simulink model "ModelBoostPFCController"  (R2026a)
settings: Solver=ode23t  StopTime=0.02  MaxStep=1e-5  AbsTol=1e-3
PreLoadFcn:
  | BoostPFCDefaultInputParameters;
model workspace (MAT data in the model file):
  ConverterKey = "BoostPFC"
undefined symbols (not defined in the file or in its folder): boostPFCController, boostPFCDesign, Vref
libraries: fl_lib x27, ee_lib x14, nesl_utility x14, ConverterLibrary x1
(part 1 of 2)
settings Model: SimulationMode=accelerator  Creator=vsolaise  LastModifiedBy=vsolaise
settings SimscapeCC: SimscapeNominalValues="[{\"value\":\"1\",\"unit\":\"A\"},{\"value\":\"1\",\"unit\":\"bar\"},{\"value\":\"1\",\"unit\":\"cm^2\"},{\"value\":\"1\",\"unit\":\"cm^3/s\"},{\"value\":\"1\",\"unit\":\"kJ/kg\"},{\"value\":\"1\",\"unit\":\"kW\"},{\"value\":\"1\",\"unit\":\"l\"},{\"value\":\"1\",\"unit\":\"N\"},{\"value\":\"1\",\"unit\":\"N*m\"},{\"value\":\"1\",\"unit\":\"V\"}]"  SimscapeLogDataHistory=5000.0

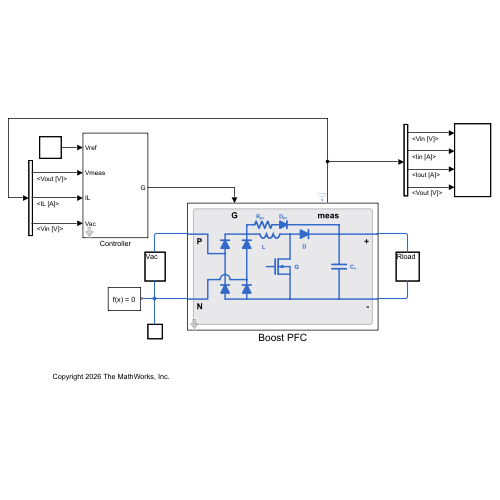
[thumbnail: Simulink's stored preview of the top-level diagram]
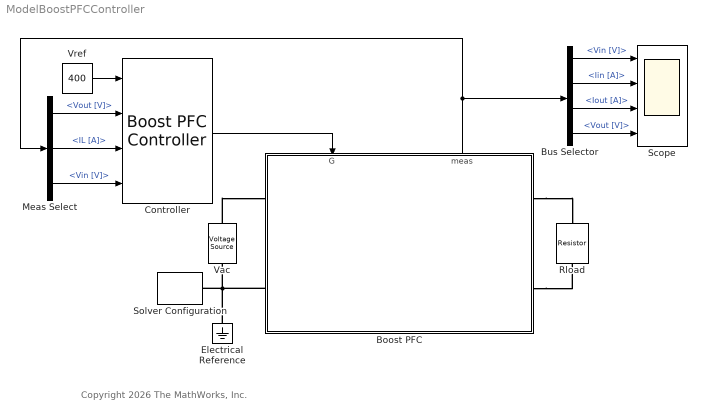
== system ModelBoostPFCController ==
  note: Copyright 2026 The MathWorks, Inc.
  Boost PFC : Subsystem  mask(Boost PFC Converter){modelOption=Simplified, ratedPower=boostPFCDesign.ratedPower.value, ratedPower_unit=W, VIn=boostPFCDesign.nomInputVoltage.value, VIn_unit=V, FRated=boostPFCDesign.lineFrequency.value, FRated_unit=Hz, VOut=boostPFCDesign.outputVoltage.value, VOut_unit=V, Fsw=boostPFCDesign.switchingFrequency.value, Fsw_unit=Hz, LBoost=boostPFCDesign.boostInductance.value, LBoost_unit=H, RLboost=boostPFCDesign.inductorResistance.value, RLboost_unit=Ohm, CBoost=2*boostPFCDesign.outputCapacitance.value, CBoost_unit=F, Rco=boostPFCDesign.capacitorResistance.value, Rco_unit=Ohm, Vco=Vref*0.95, Vco_unit=V, switchDeviceOption=MOSFET (Ideal, Switching) with Thermal, RdsOn=0.05, RdsOn_unit=Ohm, GdsOff=1e-5, GdsOff_unit=1/Ohm, Vth=3, Vth_unit=V, diodeDeviceOption=Tabulated Diode, VfDiode=0.6, VfDiode_unit=V, RdDiode=0.01, RdDiode_unit=Ohm, GdDiode=1e-5, GdDiode_unit=1/Ohm, rectDiodeDeviceOption=Tabulated Diode, VfRect=0.6, VfRect_unit=V, RdRect=0.3, RdRect_unit=Ohm, GdRect=1e-5, GdRect_unit=1/Ohm, VfPreCharge=0.6, VfPreCharge_unit=V, RdPreCharge=0.01, RdPreCharge_unit=Ohm, GdPreCharge=1e-5, GdPreCharge_unit=1/Ohm, RPreCharge=3, RPreCharge_unit=Ohm, simTemp=25, simTemp_unit=degC}
      mask prompts: modelOption "Boost PFC model option"; ratedPower "Rated power"; VIn "AC input voltage (RMS)"; FRated "Line frequency"; VOut "DC output voltage"; Fsw "Switching frequency"; LBoost "Boost inductance"; RLboost "Inductor resistance"; CBoost "Output capacitance"; Rco "Capacitor ESR"; Vco "Initial output capacitor voltage"; switchDeviceOption "Switch model"; RdsOn "On-state resistance"; GdsOff "Off-state conductance"; Vth "Threshold voltage"; diodeDeviceOption "Diode model"; VfDiode "Forward voltage"; RdDiode "On resistance"; GdDiode "Off conductance"; rectDiodeDeviceOption "Rectifier diode model"; VfRect "Forward voltage"; RdRect "On resistance"; GdRect "Off conductance"; VfPreCharge "Forward voltage"; RdPreCharge "On resistance"; GdPreCharge "Off conductance"; RPreCharge "Pre-charge resistance"; simTemp "Simulation temperature"
      mask help: Single-phase diode bridge + boost PFC power stage
      mask init:
      | %% Unit conversion: convert displayed values to base SI units
      | convMap = containers.Map( ...
      |     {'W','kW','MW','V','kV','mV','F','mF','uF','nF','pF', ...
      |      'H','mH','uH','nH','Ohm','kOhm','mOhm','S','mS','1/Ohm', ...
      |      'Hz','kHz','MHz'}, ...
      |     {1, 1e3, 1e6, 1, 1e3, 1e-3, 1, 1e-3, 1e-6, 1e-9, 1e-12, ...
      |      1, 1e-3, 1e-6, 1e-9, 1, 1e3, 1e-3, 1, 1e-3, 1, ...
      |      1, 1e3, 1e6});
      | 
      | ratedPower_SI = ratedPower * convMap(ratedPower_unit);
      | VIn_SI = VIn * convMap(VIn_unit);
      | FRated_SI = FRated * convMap(FRated_unit);
      | VOut_SI = VOut * convMap(VOut_unit);
      | Fsw_SI = Fsw * convMap(Fsw_unit);
      | LBoost_SI = LBoost * convMap(LBoost_unit);
      | RLboost_SI = RLboost * convMap(RLboost_unit);
      | CBoost_SI = CBoost * convMap(CBoost_unit);
      | Rco_SI = Rco * convMap(Rco_unit);
      | Vco_SI = Vco * convMap(Vco_unit);
      | RdsOn_SI = RdsOn * convMap(RdsOn_unit);
      | GdsOff_SI = GdsOff * convMap(GdsOff_unit);
      | Vth_SI = Vth * convMap(Vth_unit);
      | VfDiode_SI = VfDiode * convMap(VfDiode_unit);
      | RdDiode_SI = RdDiode * convMap(RdDiode_unit);
      | GdDiode_SI = GdDiode * convMap(GdDiode_unit);
      | 
      | 
      | VfRect_SI = VfRect * convMap(VfRect_unit);
      | RdRect_SI = RdRect * convMap(RdRect_unit);
      | GdRect_SI = GdRect * convMap(GdRect_unit);
      | % Pre-charge circuit parameters
      | VfPreCharge_SI = VfPreCharge * convMap(VfPreCharge_unit);
      | RdPreCharge_SI = RdPreCharge * convMap(RdPreCharge_unit);
      | GdPreCharge_SI = GdPreCharge * convMap(GdPreCharge_unit);
      | RPreCharge_SI = RPreCharge * convMap(RPreCharge_unit);
      | 
      | 
      | %% Simulation temperature (thermal MOSFET and tabulated diodes)
      | % Temperature is an OFFSET unit (K = degC + 273.15), so it cannot use the
      | % multiplicative convMap above; convert it explicitly. simTemp_K is read directly by
      | % the thermal MOSFET junction-temperature target, by the boost switch's Temperature Source, and by
      | % every tabulated diode's device simulation temperature.
      | if strcmp(simTemp_unit, 'degC')
      |     simTemp_K = simTemp + 273.15;
      | else
      |     simTemp_K = simTemp;
      | end
      | 
      | %% Apply variant selection
      | selectBoostPFCModelOption(gcb);
      settings: CopyFcn="set_param(gcbh,\"LinkStatus\",\"none\");"  PortSchema="{\"entries\":[{\"content\":{\"sides\":[{\"content\":{\"connectorIds\":[\"LConn1\",\"LConn2\"]},\"type\":\"ConnectorPlacement.EquallySpacedRectSide\",\"uuid\":\"1dbc8d27-ad96-467a-a357-3fb6b54f5038\"},{\"content\":{\"connectorIds\":[\"RConn1\",\"RConn2\"],\"side\":\"RIGHT\"},\"type\":\"ConnectorPlacement.EquallySpacedRectSide\",\"uuid\":\"a7801564-f46e-4876-bbd0-388b36974b7d\"},{\"content\":{\"connectorIds\":[\"In1\",\"Out1\"],\"side\":\"TOP\"},\"type\":\"ConnectorPlacement.EquallySpacedRectSide\",\"uuid\":\"b9e6132f-a5e8-4db3-b298-fdce73dc02b1\"}]},\"type\":\"ConnectorPlacement.EquallySpacedConnector\",\"uuid\":\"f45ea93c-581d-4ac6-a344-7b31d290ff6c\"}],\"packageUris\":[\"http://schema.mathworks.com/mf0/Connector/R2020b\"],\"version\":\"1.0\"}"
      mask Help: web('BoostPFC.html')
      mask TypeOptions modelOption: Simplified | Detailed
      mask Callback modelOption: selectBoostPFCModelOption(gcb);
      mask TypeOptions ratedPower_unit: W | kW | MW
      mask TypeOptions VIn_unit: V | kV | mV
      mask TypeOptions FRated_unit: Hz | kHz
      mask TypeOptions VOut_unit: V | kV | mV
      mask TypeOptions Fsw_unit: Hz | kHz | MHz
      mask TypeOptions LBoost_unit: H | mH | uH
      mask TypeOptions RLboost_unit: Ohm | kOhm | mOhm
      mask TypeOptions CBoost_unit: F | mF | uF | nF
      mask TypeOptions Rco_unit: Ohm | kOhm | mOhm
      mask TypeOptions Vco_unit: V | kV | mV
      mask TypeOptions switchDeviceOption: Ideal Switch | MOSFET (Ideal, Switching) with Thermal
      mask Callback switchDeviceOption: selectBoostPFCSwitchDevice(gcb);
      mask TypeOptions RdsOn_unit: Ohm | kOhm | mOhm
      mask TypeOptions GdsOff_unit: 1/Ohm | S | mS
      mask TypeOptions Vth_unit: V | kV | mV
      mask TypeOptions diodeDeviceOption: Ideal Diode | Tabulated Diode
      mask Callback diodeDeviceOption: selectBoostPFCDiodeDevice(gcb);
      mask TypeOptions VfDiode_unit: V | kV | mV
      mask TypeOptions RdDiode_unit: Ohm | kOhm | mOhm
      mask TypeOptions GdDiode_unit: 1/Ohm | S | mS
      mask TypeOptions rectDiodeDeviceOption: Ideal Diode | Tabulated Diode
      mask Callback rectDiodeDeviceOption: selectBoostPFCRectifierDiodeDevice(gcb);
      mask TypeOptions VfRect_unit: V | mV | kV
      mask TypeOptions RdRect_unit: Ohm | mOhm | kOhm
      mask TypeOptions GdRect_unit: 1/Ohm
      mask TypeOptions VfPreCharge_unit: V | kV | mV
      mask TypeOptions RdPreCharge_unit: Ohm | kOhm | mOhm
      mask TypeOptions GdPreCharge_unit: 1/Ohm | S | mS
      mask TypeOptions RPreCharge_unit: Ohm | kOhm | mOhm
      mask TypeOptions simTemp_unit: degC | K
      mask DialogControl BoostPFCConverterParameters Prompt: Boost PFC Converter Parameters
      mask DialogControl SwitchDevice Prompt: Boost Stage Devices
      mask DialogControl openMOSFETMask Prompt: Open MOSFET block mask
      mask DialogControl openMOSFETMask Callback: open_system([gcb '/BoostPFCVariant/DetailedModel/BoostSwitch/SwitchingMOSFETwithThermal/MOSFET'], 'mask');
      mask DialogControl DiodeDevice Prompt: Boost Diode Device
      mask DialogControl openDiodeMask Prompt: Open Diode block mask
      mask DialogControl openDiodeMask Callback: open_system([gcb '/BoostPFCVariant/DetailedModel/BoostDiode/TabulatedDiode/Diode1'], 'mask');
      mask DialogControl RectifierDevices Prompt: Rectifier Devices
      mask DialogControl openRectDiodeMask Prompt: Open Rectifier Diode Mask
      mask DialogControl openRectDiodeMask Callback: open_system([gcb '/BoostPFCVariant/DetailedModel/RectifierBridge/TabulatedDiode/Diode1'], 'mask');
      mask DialogControl applyRectDiodeParam Prompt: Apply to All Rectifier Diodes
      mask DialogControl applyRectDiodeParam Callback: applyBoostPFCRectifierDiodeParameters(gcb);
      mask DialogControl PreChargeCircuit Prompt: Pre-Charge Circuit Parameters
      mask DialogControl ExportPanel Prompt: Export to Unmasked Subsystem
      mask DialogControl ExportInfo Prompt: To customize the converter, export it as an unmasked subsystem with the active variant flattened - a standalone, fully-editable circuit plus a parameter file. Requires the "Variant Manager for Simulink" add-on.
      mask DialogControl exportToModel Prompt: Export
      mask DialogControl exportToModel Callback: exportConverterModelFromMask(gcb);
      mask Display: image('BoostPFCDiodeIcon.svg');
  Bus Selector : BusSelector  OutputSignals=Vin [V],Iin [A],Iout [A],Vout [V]
  Controller : ConverterLibrary/Controller/Power Factor Correction Converters/Boost PFC Controller  outputSelect=PWM Signal  cntrlSelect=PI controller (Continuous)  VacRMS=boostPFCDesign.nomInputVoltage.value  VbaseDC=boostPFCDesign.outputVoltage.value  Pbase=boostPFCDesign.ratedPower.value  PrefPu=boostPFCController.PrefPu  iRefPeakMaxPu=boostPFCController.iRefPeakMaxPu  Fsw=boostPFCDesign.switchingFrequency.value  Ts=boostPFCController.TsPwm  gateVoltageOn=boostPFCController.gateVoltageOn  gateVoltageOff=boostPFCController.gateVoltageOff  KpVoltage=boostPFCController.KpVoltage  KiVoltage=boostPFCController.KiVoltage  TsVoltage=boostPFCController.TsVoltage  KpCurrent=boostPFCController.KpCurrent  KiCurrent=boostPFCController.KiCurrent  dutyMax=boostPFCController.dutyMax  dutyMin=boostPFCController.dutyMin  TsCurrent=boostPFCController.TsCurrent
      link override Current Controller: LabelModeActiveChoice=PIContinuous
      link override Output Mode: LabelModeActiveChoice=PWMSignal
      link override Output Mode/PWMSignal/Ramp Mode: LabelModeActiveChoice=VariableStep
      link override Voltage Controller: LabelModeActiveChoice=PIContinuous
      settings: SourceProductName=Simscape Power Converter Components
  Electrical Reference : fl_lib/Electrical/Electrical Elements/Electrical Reference
  Meas Select : BusSelector  OutputSignals=Vout [V],IL [A],Vin [V]
  Rload : fl_lib/Electrical/Electrical Elements/Resistor  R=160 Ohm  i_specify=off  i_priority=None  i=0 A  i_nominal_specify=off  i_nominal_value=1  i_nominal_unit=A  v_specify=off  v_priority=None  v=0 V  v_nominal_specify=off  v_nominal_value=1  v_nominal_unit=V
  Scope : Scope  NumInputPorts=4
      settings: ActiveDisplayString=4  Title=Output Voltage (V)  ActiveDisplayYMinimum=303.40542444423374  ActiveDisplayYMaximum=409.6389638703705
  Solver Configuration : nesl_utility/Solver Configuration  PhysicalDomain=network_engine_domain  SubClassName=solver  LeftPortType=input  RightPortType=generic  Tones=[]  Harmonics=[]  SimulateNoise=off  Profile=off  UseLocalSampling=off  EnableSwitchedLinearOptims=on  FrequencyDomain=off  UseCCode=off  RelTol=0.001  AbsTol=0.001  MinStep=1e-09  ToWorkspace=off  RevertToSquareIcSolve=off  NumHomotopyIterations=100  PhasorMode=off  PhasorModeNumHarmonics=1  ConsistencySolver=NEWTON_XTOL_AFTER_FTOL  CanonicalOrdering=UNORDERED  OptimizeIntermediates=UNOPTIMIZED  IndexReductionMethod=DerivativeReplacement  DoDC=off  ResidualTolerance=1e-09  ConsistencyTolSource=GLOBAL  ConsistencyAbsTol=0.001  ConsistencyRelTol=0.001  ConsistencyTolFactor=0.001  UseLocalSolver=on  LocalSolverChoice=NE_BACKWARD_EULER_ADVANCER  ResolveIndetEquations=on  FunctionEvalNumThread=1  LocalSolverSampleTime=1/(25*boostPFCDesign.switchingFrequency.value)  DoFixedCost=off  MaxNonlinIter=3  MaxModeIter=2  ComputeImpulses=off  ImpulseIterations=2  LinearAlgebra=auto  LinearAlgebraNumThread=0  EquationFormulation=NE_TIME_EF  DelaysMemoryBudget=1024  AutomaticFiltering=on  FilteringTimeConstant=0.001  PartitionStorageMethod=AS_NEEDED  PartitionMemoryBudget=1024  PartitionMethod=ROBUST  MultibodyUseLocalSolver=off  MultibodyLocalSolverChoice=ODE1  MultibodyLocalSolverSampleTime=0.001
  Vac : ee_lib/Sources/Voltage Source  dc_voltage=0 V  ac_voltage=230*sqrt(2) V  ac_shift=0 rad  ac_frequency=50 Hz  noise_mode=ee.enum.sources.noise.Disabled  PSD=0 V^2/Hz  sample_time=1e-3 s  repeatability=ee.enum.sources.repeatability.NotRepeatable  user_seed=0  auto_seed=436666721  i_specify=off  i_priority=None  i=0 A  i_nominal_specify=off  i_nominal_value=1  i_nominal_unit=A  v_specify=off  v_priority=None  v=0 V  v_nominal_specify=off  v_nominal_value=1  v_nominal_unit=V
  Vref : Constant  Value=400
  wires:
  Boost PFC/1(meas) -> Meas Select/1, Bus Selector/1
  Vref/1 -> Controller/1
  Meas Select/1 -> Controller/2  "<Vout [V]>"
  Meas Select/2 -> Controller/3  "<IL [A]>"
  Meas Select/3 -> Controller/4  "<Vin [V]>"
  Controller/1 -> Boost PFC/1(G)
  Bus Selector/1 -> Scope/1  "<Vin [V]>"
  Bus Selector/2 -> Scope/2  "<Iin [A]>"
  Bus Selector/3 -> Scope/3  "<Iout [A]>"
  Bus Selector/4 -> Scope/4  "<Vout [V]>"
  connections:
  Vac/LConn1 -- Boost PFC/LConn1
  Boost PFC/RConn1 -- Rload/LConn1
  Boost PFC/RConn2 -- Rload/RConn1
  Electrical Reference/LConn1 -- Boost PFC/LConn2 -- Solver Configuration/RConn1 -- Vac/RConn1

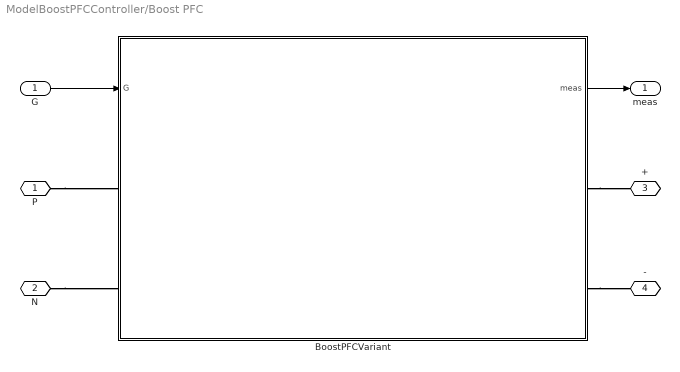
== system ModelBoostPFCController/Boost PFC ==
  G : Inport
  BoostPFCVariant : Subsystem  Variant=on  VariantControlMode=label  LabelModeActiveChoice=SimplifiedModel
  P : PMIOPort  Side=Left
  N : PMIOPort  Port=2  Side=Left
  + : PMIOPort  Port=3  Side=Right
  - : PMIOPort  Port=4  Side=Right
  meas : Outport
  wires:
  BoostPFCVariant/1(meas) -> meas/1
  G/1 -> BoostPFCVariant/1(G)
  connections:
  BoostPFCVariant/RConn2 -- -/RConn1
  BoostPFCVariant/RConn1 -- +/RConn1
  N/RConn1 -- BoostPFCVariant/LConn2
  P/RConn1 -- BoostPFCVariant/LConn1

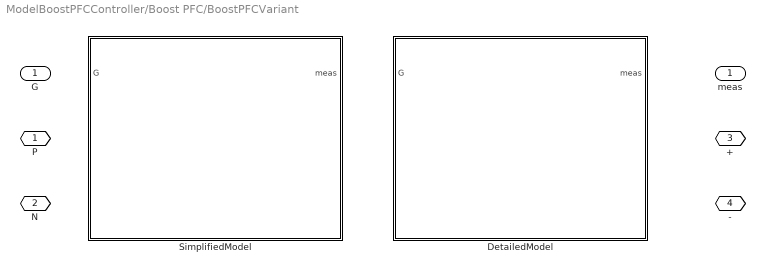
== system ModelBoostPFCController/Boost PFC/BoostPFCVariant ==
  G : Inport
  DetailedModel : Subsystem  VariantControl=DetailedModel
  SimplifiedModel : Subsystem  VariantControl=SimplifiedModel
  P : PMIOPort  Side=Left
  N : PMIOPort  Port=2  Side=Left
  + : PMIOPort  Port=3  Side=Right
  - : PMIOPort  Port=4  Side=Right
  meas : Outport

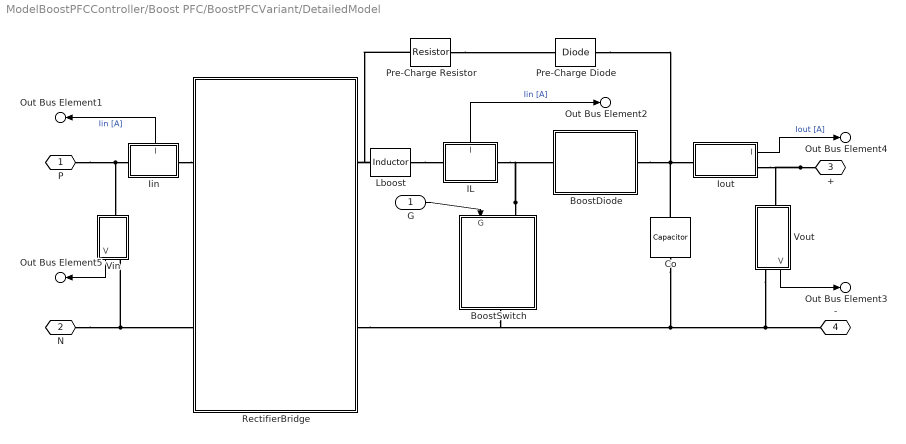
== system ModelBoostPFCController/Boost PFC/BoostPFCVariant/DetailedModel ==
  G : Inport
  BoostDiode : Subsystem  Variant=on  VariantControlMode=label  LabelModeActiveChoice=TabulatedDiode
  BoostSwitch : Subsystem  Variant=on  VariantControlMode=label  LabelModeActiveChoice=SwitchingMOSFETwithThermal
  Co : ee_lib/Passive/Capacitor  cap_option=ee.enum.passive.capacitor.capOption.const  c=CBoost_SI F  Cvec=[1e-05, 1e-06] F  Vvec=[0, 10] V  CV_table_symmetry=ee.enum.passive.capacitor.tableSymmetry.yes  f_vec=[1, 10] kHz  DFext_vec=[.8, 1.2]  enable_C_tol=ee.enum.toleranceApplication.none  averaging_period=0 s  C_tol=5  tol_distribution=ee.enum.toleranceDistribution.uniform  nSigma=4  r=Rco_SI Ohm  g=0 1/Ohm  enable_operating_limits=ee.enum.enable.no  operating_limit_action=ee.enum.passive.reportOpLim.warn  max_working_voltage_range=[-25, 25] V  power_rating=1 W  maxTemperature=85 degC  thermalEnable=false  thermalMass=1 J/K  i_specify=off  i_priority=None  i=0 A  i_nominal_specify=off  i_nominal_value=1  i_nominal_unit=A  v_specify=off  v_priority=None  v=0 V  v_nominal_specify=off  v_nominal_value=1  v_nominal_unit=V  vc_specify=on  vc_priority=High  vc=Vco_SI V  vc_nominal_specify=off  vc_nominal_value=1  vc_nominal_unit=V  T_specify=off  T_priority=None  T=298.15 K  T_nominal_specify=off  T_nominal_value=1  T_nominal_unit=K
  IL : Subsystem
      settings: PortSchema="{\"entries\":[{\"content\":{\"sides\":[{\"content\":{\"connectorIds\":[\"LConn1\"]},\"type\":\"ConnectorPlacement.EquallySpacedRectSide\",\"uuid\":\"80632e7e-66fe-49c8-894c-61cf7358e53a\"},{\"content\":{\"connectorIds\":[\"RConn1\"],\"side\":\"RIGHT\"},\"type\":\"ConnectorPlacement.EquallySpacedRectSide\",\"uuid\":\"7fb991d4-0257-47fa-8c16-238ff3f2e60c\"},{\"content\":{\"connectorIds\":[\"Out1\"],\"side\":\"TOP\"},\"type\":\"ConnectorPlacement.EquallySpacedRectSide\",\"uuid\":\"a2cf4f5e-7cb3-4577-a513-817a4fd9f07d\"}]},\"type\":\"ConnectorPlacement.EquallySpacedConnector\",\"uuid\":\"e3fac4ca-b917-4eeb-beb4-75837a4782c1\"}],\"packageUris\":[\"http://schema.mathworks.com/mf0/Connector/R2020b\"],\"version\":\"1.0\"}"
      mask Display: disp('I')
  Iin : Subsystem
      settings: PortSchema="{\"entries\":[{\"content\":{\"sides\":[{\"content\":{\"connectorIds\":[\"LConn1\"]},\"type\":\"ConnectorPlacement.EquallySpacedRectSide\",\"uuid\":\"80632e7e-66fe-49c8-894c-61cf7358e53a\"},{\"content\":{\"connectorIds\":[\"RConn1\"],\"side\":\"RIGHT\"},\"type\":\"ConnectorPlacement.EquallySpacedRectSide\",\"uuid\":\"7fb991d4-0257-47fa-8c16-238ff3f2e60c\"},{\"content\":{\"connectorIds\":[\"Out1\"],\"side\":\"TOP\"},\"type\":\"ConnectorPlacement.EquallySpacedRectSide\",\"uuid\":\"a2cf4f5e-7cb3-4577-a513-817a4fd9f07d\"}]},\"type\":\"ConnectorPlacement.EquallySpacedConnector\",\"uuid\":\"e3fac4ca-b917-4eeb-beb4-75837a4782c1\"}],\"packageUris\":[\"http://schema.mathworks.com/mf0/Connector/R2020b\"],\"version\":\"1.0\"}"
      mask Display: disp('I')
  Iout : Subsystem
      mask Display: disp('I')
  Lboost : ee_lib/Passive/Inductor  l=LBoost_SI H  enable_L_tol=ee.enum.toleranceApplication.none  L_tol=20  tol_distribution=ee.enum.toleranceDistribution.uniform  nSigma=4  r=RLboost_SI Ohm  g=1e-9 1/Ohm  enable_operating_limits=ee.enum.enable.no  operating_limit_action=ee.enum.passive.reportOpLim.warn  max_working_current=1 A  power_rating=1 W  i_L_specify=off  i_L_priority=High  i_L=0 A  i_L_nominal_specify=off  i_L_nominal_value=1  i_L_nominal_unit=A
  Pre-Charge Diode : fl_lib/Electrical/Electrical Elements/Diode  Vf=VfPreCharge_SI V  Ron=RdPreCharge_SI Ohm  Goff=GdPreCharge_SI 1/Ohm  i_specify=off  i_priority=None  i=0 A  i_nominal_specify=off  i_nominal_value=1  i_nominal_unit=A  v_specify=off  v_priority=None  v=0 V  v_nominal_specify=off  v_nominal_value=1  v_nominal_unit=V
  Pre-Charge Resistor : fl_lib/Electrical/Electrical Elements/Resistor  R=RPreCharge_SI Ohm  i_specify=off  i_priority=None  i=0 A  i_nominal_specify=off  i_nominal_value=1  i_nominal_unit=A  v_specify=off  v_priority=None  v=0 V  v_nominal_specify=off  v_nominal_value=1  v_nominal_unit=V
  RectifierBridge : Subsystem  Variant=on  VariantControlMode=label  LabelModeActiveChoice=TabulatedDiode
  Vin : Subsystem
      mask Display: disp('V')
  Vout : Subsystem
      settings: PortSchema="{\"entries\":[{\"content\":{\"sides\":[{\"content\":{\"connectorIds\":[\"LConn1\"]},\"type\":\"ConnectorPlacement.EquallySpacedRectSide\",\"uuid\":\"80632e7e-66fe-49c8-894c-61cf7358e53a\"},{\"content\":{\"connectorIds\":[\"RConn1\",\"Out1\"],\"side\":\"RIGHT\"},\"type\":\"ConnectorPlacement.EquallySpacedRectSide\",\"uuid\":\"7fb991d4-0257-47fa-8c16-238ff3f2e60c\"},{\"content\":{\"side\":\"TOP\"},\"type\":\"ConnectorPlacement.EquallySpacedRectSide\",\"uuid\":\"a2cf4f5e-7cb3-4577-a513-817a4fd9f07d\"}]},\"type\":\"ConnectorPlacement.EquallySpacedConnector\",\"uuid\":\"e3fac4ca-b917-4eeb-beb4-75837a4782c1\"}],\"packageUris\":[\"http://schema.mathworks.com/mf0/Connector/R2020b\"],\"version\":\"1.0\"}"
      mask Display: disp('V')
  P : PMIOPort  Side=Left
  N : PMIOPort  Port=2  Side=Left
  + : PMIOPort  Port=3  Side=Right
  - : PMIOPort  Port=4  Side=Right
  Out Bus Element1 : Outport  PortName=meas  Element=Iin [A]
  Out Bus Element2 : Outport  PortName=meas  Element=IL [A]
  Out Bus Element3 : Outport  PortName=meas  Element=Vout [V]
  Out Bus Element4 : Outport  PortName=meas  Element=Iout [A]
  Out Bus Element5 : Outport  PortName=meas  Element=Vin [V]
  wires:
  G/1 -> BoostSwitch/1(G)
  Iin/1(I) -> Out Bus Element1/1  "Iin [A]"
  IL/1(I) -> Out Bus Element2/1  "Iin [A]"
  Vout/1(V) -> Out Bus Element3/1
  Iout/1(I) -> Out Bus Element4/1  "Iout [A]"
  Vin/1(V) -> Out Bus Element5/1
  connections:
  Pre-Charge Resistor/RConn1 -- Pre-Charge Diode/LConn1
  P/RConn1 -- Iin/LConn1 -- Vin/LConn1
  N/RConn1 -- Vin/RConn1 -- RectifierBridge/LConn2
  Lboost/LConn1 -- Pre-Charge Resistor/LConn1 -- RectifierBridge/RConn1
  Lboost/RConn1 -- IL/LConn1
  BoostSwitch/LConn1 -- IL/RConn1 -- BoostDiode/LConn1
  BoostDiode/RConn1 -- Co/LConn1 -- Pre-Charge Diode/RConn1 -- Iout/LConn1
  +/RConn1 -- Vout/LConn1 -- Iout/RConn1
  Co/RConn1 -- -/RConn1 -- Vout/RConn1 -- RectifierBridge/RConn2 -- BoostSwitch/RConn1
  Iin/RConn1 -- RectifierBridge/LConn1

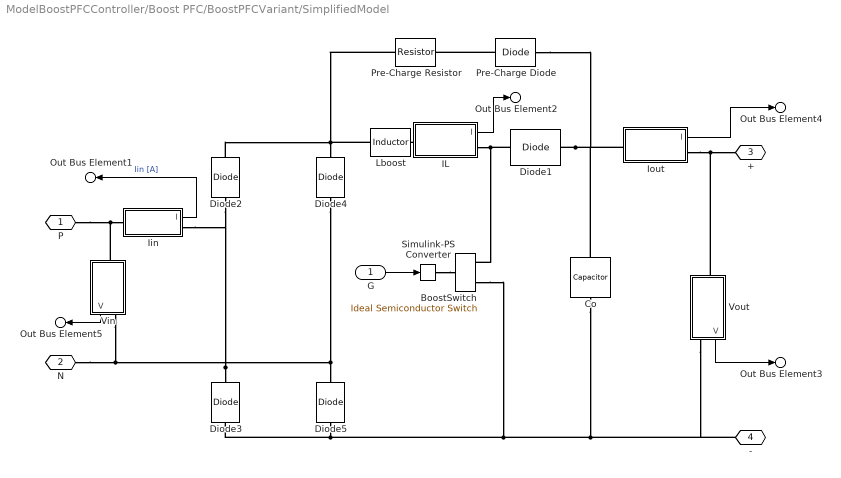
== system ModelBoostPFCController/Boost PFC/BoostPFCVariant/SimplifiedModel ==
  G : Inport
  BoostSwitch : ee_lib/Semiconductors & Converters/Ideal Semiconductor Switch  port_option=ee.enum.controlport.ps  Ron=RdsOn_SI Ohm  Goff=GdsOff_SI 1/Ohm  Vth=Vth_SI V  diode_param=ee.enum.semiconductors.protectionDiode.external  diode_Vf=0.8 V  diode_Ron=0.001 Ohm  diode_Goff=1e-5 1/Ohm  diode_C=50e-9 F  diode_iRM=-235 A  diode_iF=300 A  diode_idot=-50 A/us  diode_trr_param=ee.enum.converters.diodetrr.trr_factor  diode_trr_factor=3  diode_trr=15 us  diode_Qrr=1500 s*uA
  Co : ee_lib/Passive/Capacitor  cap_option=ee.enum.passive.capacitor.capOption.const  c=CBoost_SI F  Cvec=[1e-05, 1e-06] F  Vvec=[0, 10] V  CV_table_symmetry=ee.enum.passive.capacitor.tableSymmetry.yes  f_vec=[1, 10] kHz  DFext_vec=[.8, 1.2]  enable_C_tol=ee.enum.toleranceApplication.none  averaging_period=0 s  C_tol=5  tol_distribution=ee.enum.toleranceDistribution.uniform  nSigma=4  r=Rco_SI Ohm  g=0 1/Ohm  enable_operating_limits=ee.enum.enable.no  operating_limit_action=ee.enum.passive.reportOpLim.warn  max_working_voltage_range=[-25, 25] V  power_rating=1 W  maxTemperature=85 degC  thermalEnable=false  thermalMass=1 J/K  i_specify=off  i_priority=None  i=0 A  i_nominal_specify=off  i_nominal_value=1  i_nominal_unit=A  v_specify=off  v_priority=None  v=0 V  v_nominal_specify=off  v_nominal_value=1  v_nominal_unit=V  vc_specify=on  vc_priority=High  vc=Vco_SI V  vc_nominal_specify=off  vc_nominal_value=1  vc_nominal_unit=V  T_specify=off  T_priority=None  T=298.15 K  T_nominal_specify=off  T_nominal_value=1  T_nominal_unit=K
  Diode1 : fl_lib/Electrical/Electrical Elements/Diode  Vf=VfDiode_SI V  Ron=RdDiode_SI Ohm  Goff=GdDiode_SI 1/Ohm  i_specify=off  i_priority=None  i=0 A  i_nominal_specify=off  i_nominal_value=1  i_nominal_unit=A  v_specify=off  v_priority=None  v=0 V  v_nominal_specify=off  v_nominal_value=1  v_nominal_unit=V
  Diode{2..5} (4 alike) : fl_lib/Electrical/Electrical Elements/Diode  Vf=VfRect_SI V  Ron=RdRect_SI Ohm  Goff=GdRect_SI 1/Ohm  i_specify=off  i_priority=None  i=0 A  i_nominal_specify=off  i_nominal_value=1  i_nominal_unit=A  v_specify=off  v_priority=None  v=0 V  v_nominal_specify=off  v_nominal_value=1  v_nominal_unit=V
  IL : Subsystem
      mask Display: disp('I')
  Iin : Subsystem
      mask Display: disp('I')
  Iout : Subsystem
      mask Display: disp('I')
  Lboost : ee_lib/Passive/Inductor  l=LBoost_SI H  enable_L_tol=ee.enum.toleranceApplication.none  L_tol=20  tol_distribution=ee.enum.toleranceDistribution.uniform  nSigma=4  r=RLboost_SI Ohm  g=1e-9 1/Ohm  enable_operating_limits=ee.enum.enable.no  operating_limit_action=ee.enum.passive.reportOpLim.warn  max_working_current=1 A  power_rating=1 W  i_L_specify=off  i_L_priority=High  i_L=0 A  i_L_nominal_specify=off  i_L_nominal_value=1  i_L_nominal_unit=A
  Pre-Charge Diode : fl_lib/Electrical/Electrical Elements/Diode  Vf=VfPreCharge_SI V  Ron=RdPreCharge_SI Ohm  Goff=GdPreCharge_SI 1/Ohm  i_specify=off  i_priority=None  i=0 A  i_nominal_specify=off  i_nominal_value=1  i_nominal_unit=A  v_specify=off  v_priority=None  v=0 V  v_nominal_specify=off  v_nominal_value=1  v_nominal_unit=V
  Pre-Charge Resistor : fl_lib/Electrical/Electrical Elements/Resistor  R=RPreCharge_SI Ohm  i_specify=off  i_priority=None  i=0 A  i_nominal_specify=off  i_nominal_value=1  i_nominal_unit=A  v_specify=off  v_priority=None  v=0 V  v_nominal_specify=off  v_nominal_value=1  v_nominal_unit=V
  Simulink-PS Converter : nesl_utility/Simulink-PS Converter  PhysicalDomain=network_engine_domain  SubClassName=ps_input  LeftPortType=input  RightPortType=output  PseudoPeriodic=off  Frequencies=[]  NoiseDistribution=none  NoiseParameters=[]  Unit=1  AffineConversion=off  FilteringAndDerivatives=provide  SimscapeFilterOrder=1  InputFilterTimeConstant=0.001  UdotUserProvided=0
  Vin : Subsystem
      settings: PortSchema="{\"entries\":[{\"content\":{\"sides\":[{\"content\":{\"connectorIds\":[\"LConn1\"]},\"type\":\"ConnectorPlacement.EquallySpacedRectSide\",\"uuid\":\"5f92137b-4b58-46b8-a68f-d3527484291c\"},{\"content\":{\"connectorIds\":[\"RConn1\",\"Out1\"],\"side\":\"RIGHT\"},\"type\":\"ConnectorPlacement.EquallySpacedRectSide\",\"uuid\":\"154b36f0-aa4a-4375-80c2-9c55af429c32\"},{\"content\":{\"side\":\"TOP\"},\"type\":\"ConnectorPlacement.EquallySpacedRectSide\",\"uuid\":\"6e01dd2b-817e-4c7e-a9bf-e017a248a3a8\"}]},\"type\":\"ConnectorPlacement.EquallySpacedConnector\",\"uuid\":\"a9d15cc4-68aa-466b-9599-7a273210f999\"}],\"packageUris\":[\"http://schema.mathworks.com/mf0/Connector/R2020b\"],\"version\":\"1.0\"}"
      mask Display: disp('V')
  Vout : Subsystem
      settings: PortSchema="{\"entries\":[{\"content\":{\"sides\":[{\"content\":{\"connectorIds\":[\"LConn1\"]},\"type\":\"ConnectorPlacement.EquallySpacedRectSide\",\"uuid\":\"5f92137b-4b58-46b8-a68f-d3527484291c\"},{\"content\":{\"connectorIds\":[\"RConn1\",\"Out1\"],\"side\":\"RIGHT\"},\"type\":\"ConnectorPlacement.EquallySpacedRectSide\",\"uuid\":\"154b36f0-aa4a-4375-80c2-9c55af429c32\"},{\"content\":{\"side\":\"TOP\"},\"type\":\"ConnectorPlacement.EquallySpacedRectSide\",\"uuid\":\"6e01dd2b-817e-4c7e-a9bf-e017a248a3a8\"}]},\"type\":\"ConnectorPlacement.EquallySpacedConnector\",\"uuid\":\"a9d15cc4-68aa-466b-9599-7a273210f999\"}],\"packageUris\":[\"http://schema.mathworks.com/mf0/Connector/R2020b\"],\"version\":\"1.0\"}"
      mask Display: disp('V')
  P : PMIOPort  Side=Left
  N : PMIOPort  Port=2  Side=Left
  + : PMIOPort  Port=3  Side=Right
  - : PMIOPort  Port=4  Side=Right
  Out Bus Element1 : Outport  PortName=meas  Element=Iin [A]
  Out Bus Element2 : Outport  PortName=meas  Element=IL [A]
  Out Bus Element3 : Outport  PortName=meas  Element=Vout [V]
  Out Bus Element4 : Outport  PortName=meas  Element=Iout [A]
  Out Bus Element5 : Outport  PortName=meas  Element=Vin [V]
  wires:
  Vin/1(V) -> Out Bus Element5/1
  IL/1(I) -> Out Bus Element2/1
  Vout/1(V) -> Out Bus Element3/1
  Iout/1(I) -> Out Bus Element4/1
  Iin/1(I) -> Out Bus Element1/1  "Iin [A]"
  G/1 -> Simulink-PS Converter/1
  connections:
  Pre-Charge Diode/LConn1 -- Pre-Charge Resistor/RConn1
  Iin/LConn1 -- Vin/LConn1 -- P/RConn1
  Diode2/RConn1 -- Lboost/LConn1 -- Pre-Charge Resistor/LConn1 -- Diode4/RConn1
  Diode3/RConn1 -- Iin/RConn1 -- Diode2/LConn1
  Vin/RConn1 -- Diode4/LConn1 -- Diode5/RConn1 -- N/RConn1
  Diode5/LConn1 -- Vout/RConn1 -- -/RConn1 -- Co/RConn1 -- BoostSwitch/RConn2 -- Diode3/LConn1
  Diode1/LConn1 -- IL/RConn1 -- BoostSwitch/RConn1
  Simulink-PS Converter/RConn1 -- BoostSwitch/LConn1
  Diode1/RConn1 -- Co/LConn1 -- Pre-Charge Diode/RConn1 -- Iout/LConn1
  IL/LConn1 -- Lboost/RConn1
  Iout/RConn1 -- Vout/LConn1 -- +/RConn1

== system ModelBoostPFCController/Boost PFC/BoostPFCVariant/DetailedModel/BoostDiode ==
  IdealDiode : Subsystem  VariantControl=IdealDiode
  TabulatedDiode : Subsystem  VariantControl=TabulatedDiode
  A : PMIOPort  Side=Left
  K : PMIOPort  Port=2  Side=Right

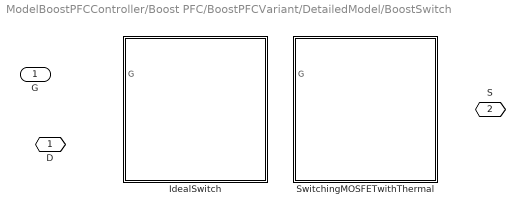
== system ModelBoostPFCController/Boost PFC/BoostPFCVariant/DetailedModel/BoostSwitch ==
  G : Inport
  IdealSwitch : Subsystem  VariantControl=IdealSwitch
  SwitchingMOSFETwithThermal : Subsystem  VariantControl=SwitchingMOSFETwithThermal
  D : PMIOPort  Side=Left
  S : PMIOPort  Port=2  Side=Right

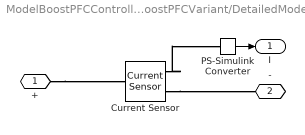
== system ModelBoostPFCController/Boost PFC/BoostPFCVariant/DetailedModel/IL ==
  Current Sensor : fl_lib/Electrical/Electrical Sensors/Current Sensor
  PS-Simulink Converter : nesl_utility/PS-Simulink Converter  PhysicalDomain=network_engine_domain  SubClassName=ps_output  LeftPortType=input  RightPortType=output  PseudoPeriodic=off  Frequencies=[]  VectorFormat=inherit  Unit=inherit  AffineConversion=off
  + : PMIOPort  Side=Left
  - : PMIOPort  Port=2  Side=Right
  I : Outport
  wires:
  PS-Simulink Converter/1 -> I/1
  connections:
  Current Sensor/RConn1 -- PS-Simulink Converter/LConn1
  Current Sensor/RConn2 -- -/RConn1
  +/RConn1 -- Current Sensor/LConn1

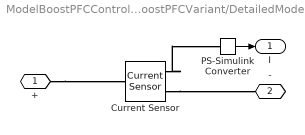
== system ModelBoostPFCController/Boost PFC/BoostPFCVariant/DetailedModel/Iin ==
  Current Sensor : fl_lib/Electrical/Electrical Sensors/Current Sensor
  PS-Simulink Converter : nesl_utility/PS-Simulink Converter  PhysicalDomain=network_engine_domain  SubClassName=ps_output  LeftPortType=input  RightPortType=output  PseudoPeriodic=off  Frequencies=[]  VectorFormat=inherit  Unit=inherit  AffineConversion=off
  + : PMIOPort  Side=Left
  - : PMIOPort  Port=2  Side=Right
  I : Outport
  wires:
  PS-Simulink Converter/1 -> I/1
  connections:
  Current Sensor/RConn1 -- PS-Simulink Converter/LConn1
  Current Sensor/RConn2 -- -/RConn1
  +/RConn1 -- Current Sensor/LConn1

== system ModelBoostPFCController/Boost PFC/BoostPFCVariant/DetailedModel/Iout ==
  Current Sensor : fl_lib/Electrical/Electrical Sensors/Current Sensor
  PS-Simulink Converter : nesl_utility/PS-Simulink Converter  PhysicalDomain=network_engine_domain  SubClassName=ps_output  LeftPortType=input  RightPortType=output  PseudoPeriodic=off  Frequencies=[]  VectorFormat=inherit  Unit=inherit  AffineConversion=off
  + : PMIOPort  Side=Left
  - : PMIOPort  Port=2  Side=Right
  I : Outport
  wires:
  PS-Simulink Converter/1 -> I/1
  connections:
  Current Sensor/RConn1 -- PS-Simulink Converter/LConn1
  Current Sensor/RConn2 -- -/RConn1
  +/RConn1 -- Current Sensor/LConn1

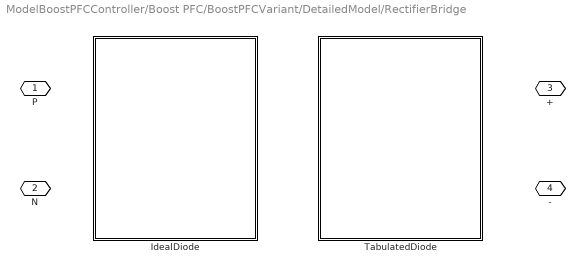
== system ModelBoostPFCController/Boost PFC/BoostPFCVariant/DetailedModel/RectifierBridge ==
  IdealDiode : Subsystem  VariantControl=IdealDiode
  TabulatedDiode : Subsystem  VariantControl=TabulatedDiode
  P : PMIOPort  Side=Left
  N : PMIOPort  Port=2  Side=Left
  + : PMIOPort  Port=3  Side=Right
  - : PMIOPort  Port=4  Side=Right

== system ModelBoostPFCController/Boost PFC/BoostPFCVariant/DetailedModel/Vin ==
  PS-Simulink Converter : nesl_utility/PS-Simulink Converter  PhysicalDomain=network_engine_domain  SubClassName=ps_output  LeftPortType=input  RightPortType=output  PseudoPeriodic=off  Frequencies=[]  VectorFormat=inherit  Unit=inherit  AffineConversion=off
  Voltage Sensor : fl_lib/Electrical/Electrical Sensors/Voltage Sensor
  + : PMIOPort  Side=Left
  - : PMIOPort  Port=2  Side=Right
  V : Outport
  wires:
  PS-Simulink Converter/1 -> V/1
  connections:
  Voltage Sensor/RConn1 -- PS-Simulink Converter/LConn1
  Voltage Sensor/RConn2 -- -/RConn1
  +/RConn1 -- Voltage Sensor/LConn1

== system ModelBoostPFCController/Boost PFC/BoostPFCVariant/DetailedModel/Vout ==
  PS-Simulink Converter : nesl_utility/PS-Simulink Converter  PhysicalDomain=network_engine_domain  SubClassName=ps_output  LeftPortType=input  RightPortType=output  PseudoPeriodic=off  Frequencies=[]  VectorFormat=inherit  Unit=inherit  AffineConversion=off
  Voltage Sensor : fl_lib/Electrical/Electrical Sensors/Voltage Sensor
  + : PMIOPort  Side=Left
  - : PMIOPort  Port=2  Side=Right
  V : Outport
  wires:
  PS-Simulink Converter/1 -> V/1
  connections:
  Voltage Sensor/RConn1 -- PS-Simulink Converter/LConn1
  Voltage Sensor/RConn2 -- -/RConn1
  +/RConn1 -- Voltage Sensor/LConn1

== system ModelBoostPFCController/Boost PFC/BoostPFCVariant/SimplifiedModel/IL ==
  Current Sensor : fl_lib/Electrical/Electrical Sensors/Current Sensor
  PS-Simulink Converter : nesl_utility/PS-Simulink Converter  PhysicalDomain=network_engine_domain  SubClassName=ps_output  LeftPortType=input  RightPortType=output  PseudoPeriodic=off  Frequencies=[]  VectorFormat=inherit  Unit=inherit  AffineConversion=off
  + : PMIOPort  Side=Left
  - : PMIOPort  Port=2  Side=Right
  I : Outport
  wires:
  PS-Simulink Converter/1 -> I/1
  connections:
  Current Sensor/RConn1 -- PS-Simulink Converter/LConn1
  Current Sensor/RConn2 -- -/RConn1
  +/RConn1 -- Current Sensor/LConn1

== system ModelBoostPFCController/Boost PFC/BoostPFCVariant/SimplifiedModel/Iin ==
  Current Sensor : fl_lib/Electrical/Electrical Sensors/Current Sensor
  PS-Simulink Converter : nesl_utility/PS-Simulink Converter  PhysicalDomain=network_engine_domain  SubClassName=ps_output  LeftPortType=input  RightPortType=output  PseudoPeriodic=off  Frequencies=[]  VectorFormat=inherit  Unit=inherit  AffineConversion=off
  + : PMIOPort  Side=Left
  - : PMIOPort  Port=2  Side=Right
  I : Outport
  wires:
  PS-Simulink Converter/1 -> I/1
  connections:
  +/RConn1 -- Current Sensor/LConn1
  Current Sensor/RConn2 -- -/RConn1
  Current Sensor/RConn1 -- PS-Simulink Converter/LConn1

== system ModelBoostPFCController/Boost PFC/BoostPFCVariant/SimplifiedModel/Iout ==
  Current Sensor : fl_lib/Electrical/Electrical Sensors/Current Sensor
  PS-Simulink Converter : nesl_utility/PS-Simulink Converter  PhysicalDomain=network_engine_domain  SubClassName=ps_output  LeftPortType=input  RightPortType=output  PseudoPeriodic=off  Frequencies=[]  VectorFormat=inherit  Unit=inherit  AffineConversion=off
  + : PMIOPort  Side=Left
  - : PMIOPort  Port=2  Side=Right
  I : Outport
  wires:
  PS-Simulink Converter/1 -> I/1
  connections:
  Current Sensor/RConn1 -- PS-Simulink Converter/LConn1
  Current Sensor/RConn2 -- -/RConn1
  +/RConn1 -- Current Sensor/LConn1

== system ModelBoostPFCController/Boost PFC/BoostPFCVariant/SimplifiedModel/Vin ==
  PS-Simulink Converter : nesl_utility/PS-Simulink Converter  PhysicalDomain=network_engine_domain  SubClassName=ps_output  LeftPortType=input  RightPortType=output  PseudoPeriodic=off  Frequencies=[]  VectorFormat=inherit  Unit=inherit  AffineConversion=off
  Voltage Sensor : fl_lib/Electrical/Electrical Sensors/Voltage Sensor
  + : PMIOPort  Side=Left
  - : PMIOPort  Port=2  Side=Right
  V : Outport
  wires:
  PS-Simulink Converter/1 -> V/1
  connections:
  +/RConn1 -- Voltage Sensor/LConn1
  Voltage Sensor/RConn2 -- -/RConn1
  Voltage Sensor/RConn1 -- PS-Simulink Converter/LConn1

== system ModelBoostPFCController/Boost PFC/BoostPFCVariant/SimplifiedModel/Vout ==
  PS-Simulink Converter : nesl_utility/PS-Simulink Converter  PhysicalDomain=network_engine_domain  SubClassName=ps_output  LeftPortType=input  RightPortType=output  PseudoPeriodic=off  Frequencies=[]  VectorFormat=inherit  Unit=inherit  AffineConversion=off
  Voltage Sensor : fl_lib/Electrical/Electrical Sensors/Voltage Sensor
  + : PMIOPort  Side=Left
  - : PMIOPort  Port=2  Side=Right
  V : Outport
  wires:
  PS-Simulink Converter/1 -> V/1
  connections:
  Voltage Sensor/RConn1 -- PS-Simulink Converter/LConn1
  Voltage Sensor/RConn2 -- -/RConn1
  +/RConn1 -- Voltage Sensor/LConn1

== system ModelBoostPFCController/Boost PFC/BoostPFCVariant/DetailedModel/BoostDiode/IdealDiode ==
  Diode1 : fl_lib/Electrical/Electrical Elements/Diode  Vf=VfDiode_SI V  Ron=RdDiode_SI Ohm  Goff=GdDiode_SI 1/Ohm  i_specify=off  i_priority=None  i=0 A  i_nominal_specify=off  i_nominal_value=1  i_nominal_unit=A  v_specify=off  v_priority=None  v=0 V  v_nominal_specify=off  v_nominal_value=1  v_nominal_unit=V
  A : PMIOPort  Side=Left
  K : PMIOPort  Port=2  Side=Right
  connections:
  Diode1/RConn1 -- K/RConn1
  A/RConn1 -- Diode1/LConn1

== system ModelBoostPFCController/Boost PFC/BoostPFCVariant/DetailedModel/BoostDiode/TabulatedDiode ==
  Diode1 : ee_lib/Semiconductors & Converters/Diode  PartSpecification="{\"CollectionId\":\"SimscapeElectrical\",\"CollectionVersion\":\"1.0.0\",\"DatasetId\":\"Infineon|IDW80C65D1|simscape.electrical.diode\",\"DisplayName\":\"Infineon:IDW80C65D1\"}"  ModelType=ee.enum.diode.modelType.tabulated  TableType=ee.enum.diode.tableType.IfMat  IfMat=[0.0001 0.0001 0.1601 0.6065 1.9426 5.4603 12.2546 21.9425 34.4556 49.1982 64.7538 83.3404;0.3114 0.8503 2.3479 5.2232 9.8335 15.9488 23.5801 32.5233 43.1998 54.3228 66.653 79.8979] % Datasheet derived A  VfMat=[.9, 1.15, 1.25, 1.5, 1.75, 2.17, 2.6, 2.85; .58, .68, .75, 1.1, 1.38, 1.77, 2.27, 2.7] % Parameter not set V  TjVec=[25 175] % Datasheet derived degC  VfVec=[0.3258 0.4465 0.5672 0.6878 0.8085 0.9292 1.0498 1.1705 1.2912 1.4118 1.5325 1.6532] % Datasheet derived V  IfVec=[.1, .2, .5, 1, 2, 4, 7, 10] % Parameter not set A  IrMat=[1e-06, 2e-06, 5e-06, 1e-05, 2.5e-05, 5e-05, .0001; 2e-06, 5e-06, 1e-05, 4e-05, 8e-05, .0002, .0005] % Parameter not set A  VrMat=[10, 100, 200, 250, 300, 325, 350; 10, 70, 160, 220, 270, 300, 320] % Parameter not set V  VrVec=[10, 20, 40, 50, 70, 80, 100] % Parameter not set V  IrVec=[1e-06, 2e-06, 5e-06, 1e-05, 2e-05, 5e-05, .0001] % Parameter not set A  Vf=0.6 % Parameter not set V  Ron=0.3 % Parameter not set Ohm  Goff=1e-08 % Parameter not set S  prmExp=ee.enum.diode.expParam.useTwo  I12=[.0137, .545] % Parameter not set A  V12=[.6, .7] % Parameter not set V  RS=0 % Parameter not set Ohm  Tmeas=298.15 % Parameter not set K  IS=1e-12 % Parameter not set A  ec=1 % Parameter not set  I1=0.0137 % Parameter not set A  V1=0.6 % Parameter not set V  N_series=1 % Parameter not set  N_parallel=1 % Parameter not set  ZenerEnable=false % Parameter not set  Rz=0.3 % Parameter not set Ohm  BV=inf % Parameter not set V  C_param=ee.enum.diode.capParam.fixed  CJ=0 % Parameter not set pF  CJ0=5 % Parameter not set pF  Vvec=[.1, 10, 100] % Parameter not set V  Cvec=[3.5, 1, .4] % Parameter not set pF  VJ=1 % Parameter not set V  Mgrad=0.5 % Parameter not set  FC=0.5 % Parameter not set  Q_param=ee.enum.diode.recoveryParam.off  iRM=-7.15 % Parameter not set A  iF=4 % Parameter not set A  didt=-750 % Parameter not set A/us  trr_factor=3 % Parameter not set  trr=115 % Parameter not set ns  Qrr=150 % Parameter not set nA*s  Vr=-600 % Parameter not set V  Ls=150 % Parameter not set nH  Erec=0.03 % Parameter not set J  TT=50 % Parameter not set ns  tau=100 % Parameter not set ns  T_param=ee.enum.diode.temperatureParam.off  Tdevice=simTemp_K K  I1_T2=0.245 % Parameter not set A  V1_T2=0.5 % Parameter not set V  IS_T2=1.25e-7 % Parameter not set A  Tmeas2=125 % Parameter not set degC  XTI_param=ee.enum.diode.xtiParam.pn  XTI=3 % Parameter not set  EG_param=ee.enum.diode.egapParam.material_si  EG=1.11 % Parameter not set eV  dBVdT=0 % Parameter not set V/K  enable_fault_input=simscape.enum.onoff.off  i_specify=off  i_priority=None  i=0 A  i_nominal_specify=off  i_nominal_value=1  i_nominal_unit=A  v_specify=off  v_priority=None  v=0 V  v_nominal_specify=off  v_nominal_value=1  v_nominal_unit=V  v_capacitor_specify=off  v_capacitor_priority=None  v_capacitor=0 V  v_capacitor_nominal_specify=off  v_capacitor_nominal_value=1  v_capacitor_nominal_unit=V  Qj_specify=off  Qj_priority=High  Qj=0 C  Qj_nominal_specify=off  Qj_nominal_value=1  Qj_nominal_unit=C  i_diode_specify=off  i_diode_priority=None  i_diode=0 A  i_diode_nominal_specify=off  i_diode_nominal_value=1  i_diode_nominal_unit=A  v_diode_specify=off  v_diode_priority=None  v_diode=0 V  v_diode_nominal_specify=off  v_diode_nominal_value=1  v_diode_nominal_unit=V  i_capacitor_specify=off  i_capacitor_priority=None  i_capacitor=0 A  i_capacitor_nominal_specify=off  i_capacitor_nominal_value=1  i_capacitor_nominal_unit=A  fidelity_level=ee.enum.diode.fidelity.includeChargeDyn  rec_loss_model=ee.enum.diode.reverseRecoveryModel.fixed  ErecVal=0 % Parameter not set J  scaleWithIandV=true % Parameter not set  ErecMat=zeros(2, 3) % Parameter not set J  ErecMat3D=zeros(2, 3, 2) J  TjrecVec=[298.15, 398.15] % Parameter not set K  IfrecVec=[.1, 1, 10] % Parameter not set A  IrecVal=10 % Parameter not set A  VrecVal=10 % Parameter not set V  VrecVec=[0, 100] V  tFilter=1 / 1000 / 100 % Parameter not set s  thermal_network_parameterization=ee.enum.thermalNetworkTopology.junctionCase  Rth=[0, 10] % Parameter not set K/W  Rth_Cauer=[1, 3, 10] % Parameter not set K/W  Rth_Foster=[.08, .14, .22, .16] % Parameter not set K/W  thermal_mass_parameterization=ee.enum.thermalNetwork.timeconstant  thermal_mass=[0, 1] % Parameter not set J/K  thermal_mass_Cauer=[.1, .3, 1] % Parameter not set J/K  thermal_mass_Foster=[.001, .005, .05, .5] % Parameter not set J/K  thermal_time_constant=[0, 10] % Parameter not set s  thermal_time_constant_Cauer=[1, 3, 10] % Parameter not set s  thermal_time_constant_Foster=[7e-05, .0007, .01, .08] % Parameter not set s  thermal_mass_initial_temperatures=[25, 25] % Parameter not set degC  thermal_mass_initial_temperatures_Cauer=[25, 25, 25] % Parameter not set degC  junction_thermal_mass=0.01 % Parameter not set J/K  Tvec_initial_Foster=[25, 25, 25, 25] % Parameter not set degC  no_thermal_network=0 % Parameter not set  junction_temperature_specify=off  junction_temperature_priority=None  junction_temperature=25 degC  junction_temperature_nominal_specify=off  junction_temperature_nominal_value=1  junction_temperature_nominal_unit=degC
      settings: AttributesFormatString=Infineon:IDW80C65D1
  A : PMIOPort  Side=Left
  K : PMIOPort  Port=2  Side=Right
  connections:
  Diode1/RConn1 -- K/RConn1
  A/RConn1 -- Diode1/LConn1

== system ModelBoostPFCController/Boost PFC/BoostPFCVariant/DetailedModel/BoostSwitch/IdealSwitch ==
  G : Inport
  MOSFET : ee_lib/Semiconductors & Converters/Ideal Semiconductor Switch  port_option=ee.enum.controlport.ps  Ron=RdsOn_SI Ohm  Goff=GdsOff_SI 1/Ohm  Vth=Vth_SI V  diode_param=ee.enum.semiconductors.protectionDiode.external  diode_Vf=0.8 V  diode_Ron=0.001 Ohm  diode_Goff=1e-5 1/Ohm  diode_C=50e-9 F  diode_iRM=-235 A  diode_iF=300 A  diode_idot=-50 A/us  diode_trr_param=ee.enum.converters.diodetrr.trr_factor  diode_trr_factor=3  diode_trr=15 us  diode_Qrr=1500 s*uA
  SL_PS : nesl_utility/Simulink-PS Converter  PhysicalDomain=network_engine_domain  SubClassName=ps_input  LeftPortType=input  RightPortType=output  PseudoPeriodic=off  Frequencies=[]  NoiseDistribution=none  NoiseParameters=[]  Unit=1  AffineConversion=off  FilteringAndDerivatives=provide  SimscapeFilterOrder=1  InputFilterTimeConstant=0.001  UdotUserProvided=0
  D : PMIOPort  Side=Left
  S : PMIOPort  Port=2  Side=Right
  wires:
  G/1 -> SL_PS/1
  connections:
  MOSFET/RConn2 -- S/RConn1
  D/RConn1 -- MOSFET/RConn1
  SL_PS/RConn1 -- MOSFET/LConn1
